simulink model "MotorDriveUnit_Component_harness_model"  (R2023a)
settings: Solver=daessc  StartTime=0.0  StopTime=600  RelTol=1e-3
PreLoadFcn:
  | MotorDriveUnit_Component_harness_params
undefined symbols (not defined in the file or in its folder): batteryHighVoltage, initial, Minus, motorDriveUnit, Plus
libraries: fl_lib x24, nesl_utility x11, sdl_lib x1
settings Model: Creator=isaacito  LastModifiedBy=isaacito
settings DataIOCC: DSMLogging=off
settings OptimizationCC: ReuseModelBlockBuffer=off
settings ModelReferenceCC: EnableRefExpFcnMdlSchedulingChecks=on
settings SimscapeCC: SimscapeLogType=all  SimscapeLogSimulationStatistics=on  SimscapeLogLimitData=off

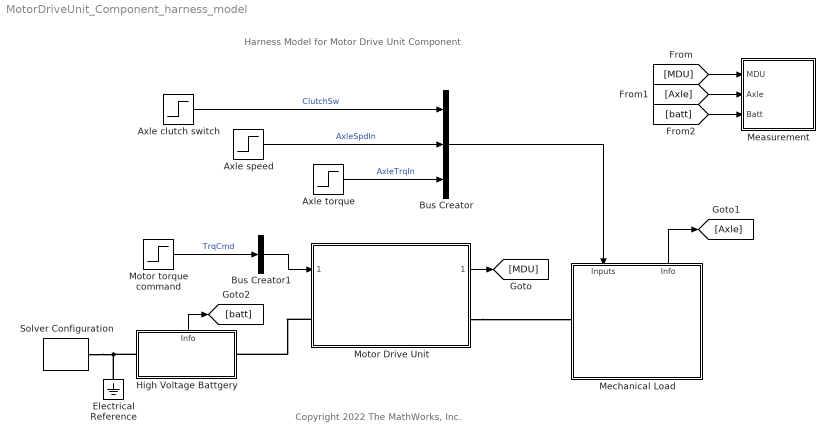
== system MotorDriveUnit_Component_harness_model ==
  note: Harness Model for Motor Drive Unit Component
  note: Copyright 2022 The MathWorks, Inc.
  Axle clutch switch : Step  After=0  SampleTime=0
      settings: AttributesFormatString=|
      | Before %<Before>
      | Time %<Time>
      | After %<After>
  Axle speed : Step  After=0  SampleTime=0
      settings: AttributesFormatString=|
      | Before %<Before>
      | Time %<Time>
      | After %<After>
  Axle torque : Step  Time=400  Before=-10  After=0  SampleTime=0
      settings: AttributesFormatString=|
      | Before %<Before>
      | Time %<Time>
      | After %<After>
  Bus Creator : BusCreator  Inputs=3
  Bus Creator1 : BusCreator  Inputs=1
  Electrical Reference : fl_lib/Electrical/Electrical Elements/Electrical Reference
  High Voltage Battgery : Subsystem
      settings: PortSchema="{\"entries\":[{\"content\":{\"sides\":[{\"content\":{\"connectorIds\":[\"LConn1\"]},\"type\":\"ConnectorPlacement.EquallySpacedRectSide\",\"uuid\":\"8acd7e9a-bb08-4de6-aa14-0989ebba81b9\"},{\"content\":{\"connectorIds\":[\"RConn1\"],\"side\":\"RIGHT\"},\"type\":\"ConnectorPlacement.EquallySpacedRectSide\",\"uuid\":\"f80e1afc-966f-4d6b-84f9-f0b60dd6f20c\"},{\"content\":{\"connectorIds\":[\"Out1\"],\"side\":\"TOP\"},\"type\":\"ConnectorPlacement.EquallySpacedRectSide\",\"uuid\":\"52ccb2b1-bd5e-4dcb-b9b6-0ef03b912c33\"}]},\"type\":\"ConnectorPlacement.EquallySpacedConnector\",\"uuid\":\"b55f48a4-f283-4a77-8513-99b31abb285a\"}],\"packageUris\":[\"http://schema.mathworks.com/mf0/Connector/R2020b\"],\"version\":\"1.0\"}"
  Measurement : Subsystem
  Mechanical Load : Subsystem
      settings: PortSchema="{\"entries\":[{\"content\":{\"sides\":[{\"content\":{\"connectorIds\":[\"LConn1\"]},\"type\":\"ConnectorPlacement.EquallySpacedRectSide\",\"uuid\":\"18221845-08ef-4cf2-b090-320221152030\"},{\"content\":{\"connectorIds\":[],\"side\":\"RIGHT\"},\"type\":\"ConnectorPlacement.EquallySpacedRectSide\",\"uuid\":\"d5b0548b-74c8-455a-9783-7dc299f3571f\"},{\"content\":{\"connectorIds\":[\"In1\",\"Out1\"],\"side\":\"TOP\"},\"type\":\"ConnectorPlacement.EquallySpacedRectSide\",\"uuid\":\"542d8e55-6d7f-4c9a-9fdc-66897ed9f466\"}]},\"type\":\"ConnectorPlacement.EquallySpacedConnector\",\"uuid\":\"3cd4c536-0337-4305-a842-969bfb1fefe3\"}],\"packageUris\":[\"http://schema.mathworks.com/mf0/Connector/R2020b\"],\"version\":\"1.0\"}"
  Motor Drive Unit : Subsystem  ReferencedSubsystem=MotorDriveUnit_refsub_Basic  torque_max=motorDriveUnit.trqMax_Nm  Value=motorDriveUnit.powerMax_kW  Tc=motorDriveUnit.responseTime_s  eff=motorDriveUnit.efficiency_pct  w_eff=motorDriveUnit.spd_eff_rpm  T_eff=motorDriveUnit.trq_eff_Nm  thermal_mass=motorDriveUnit.thermalMass_J_perK  temperature=initial.MDU_Temperature_K  k=motorDriveUnit.dampSpringStiffness_Nm_per_rad  mu_visc=motorDriveUnit.dampSpringFriction_Nm_per_rpm  w_tol=smoothing.MDU_dampSpringVelTol_rpm  T=initial.MDU_AirTemp_K
      settings: PortSchema="{\"entries\":[{\"content\":{\"sides\":[{\"content\":{\"connectorIds\":[\"In1\",\"LConn1\"]},\"type\":\"ConnectorPlacement.EquallySpacedRectSide\",\"uuid\":\"02d16a10-ccfb-4288-a5a1-1144159c5ca2\"},{\"content\":{\"connectorIds\":[\"Out1\",\"LConn2\"],\"side\":\"RIGHT\"},\"type\":\"ConnectorPlacement.EquallySpacedRectSide\",\"uuid\":\"b2601986-efe5-4f5e-bd54-3f5cb03e9252\"},{\"content\":{\"side\":\"TOP\"},\"type\":\"ConnectorPlacement.EquallySpacedRectSide\",\"uuid\":\"248805f0-4416-4f49-8b0b-c2d3fe77e89e\"}]},\"type\":\"ConnectorPlacement.EquallySpacedConnector\",\"uuid\":\"35449164-35fe-478e-9b2e-66e853caa6da\"}],\"packageUris\":[\"http://schema.mathworks.com/mf0/Connector/R2020b\"],\"version\":\"1.0\"}"
  Motor torque command : Step  Time=300  Before=150  After=-50  SampleTime=0
      settings: AttributesFormatString=|
      | Before %<Before>
      | Time %<Time>
      | After %<After>
  Solver Configuration : nesl_utility/Solver Configuration  PhysicalDomain=network_engine_domain  SubClassName=solver  LeftPortType=input  RightPortType=generic  Tones=[]  Harmonics=[]  SimulateNoise=off  Profile=off  UseLocalSampling=off  EnableSwitchedLinearOptims=on  FrequencyDomain=off  UseCCode=off  RelTol=0.001  AbsTol=1e-06  MinStep=1e-09  ToWorkspace=off  RevertToSquareIcSolve=off  NumHomotopyIterations=100  PhasorMode=off  PhasorModeNumHarmonics=1  ConsistencySolver=NEWTON_FTOL  IndexReductionMethod=DerivativeReplacement  DoDC=off  ResidualTolerance=1e-09  ConsistencyTolSource=GLOBAL  ConsistencyAbsTol=0.001  ConsistencyRelTol=0.001  ConsistencyTolFactor=0.001  UseLocalSolver=off  LocalSolverChoice=NE_BACKWARD_EULER_ADVANCER  ResolveIndetEquations=on  FunctionEvalNumThread=1  LocalSolverSampleTime=0.001  DoFixedCost=off  MaxNonlinIter=3  MaxModeIter=2  ComputeImpulses=off  ImpulseIterations=2  LinearAlgebra=auto  LinearAlgebraNumThread=0  EquationFormulation=NE_TIME_EF  DelaysMemoryBudget=1024  AutomaticFiltering=on  FilteringTimeConstant=0.001  PartitionStorageMethod=AS_NEEDED  PartitionMemoryBudget=1024  PartitionMethod=ROBUST
      settings: AttributesFormatString=Local solver %<UseLocalSolver>
  wires:
  Axle speed/1 -> Bus Creator/2  "AxleSpdIn"
  Axle torque/1 -> Bus Creator/3  "AxleTrqIn"
  Motor Drive Unit/1 -> [MDU]
  [MDU] -> Measurement/1(MDU)
  Motor torque command/1 -> Bus Creator1/1  "TrqCmd"
  Bus Creator1/1 -> Motor Drive Unit/1
  [Axle] -> Measurement/2(Axle)
  High Voltage Battgery/1(Info) -> [batt]
  [batt] -> Measurement/3(Batt)
  Bus Creator/1 -> Mechanical Load/1(Inputs)
  Mechanical Load/1(Info) -> [Axle]
  Axle clutch switch/1 -> Bus Creator/1  "ClutchSw"
  connections:
  Motor Drive Unit/LConn1 -- High Voltage Battgery/RConn1
  Electrical Reference/LConn1 -- High Voltage Battgery/LConn1 -- Solver Configuration/RConn1
  Motor Drive Unit/LConn2 -- Mechanical Load/LConn1

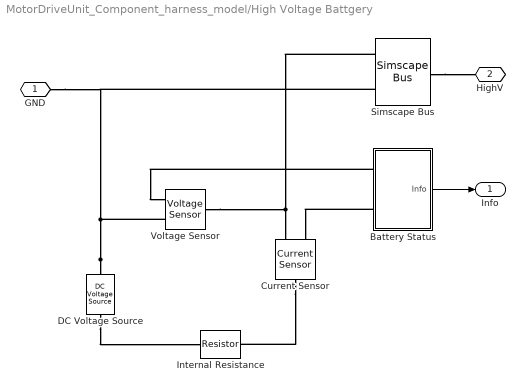
== system MotorDriveUnit_Component_harness_model/High Voltage Battgery ==
  Battery Status : Subsystem
  Current Sensor : fl_lib/Electrical/Electrical Sensors/Current Sensor
  DC Voltage Source : fl_lib/Electrical/Electrical Sources/DC Voltage Source  v0=batteryHighVoltage.voltage_V V
      settings: AttributesFormatString=%<v0> [%<v0_unit>]
  Internal Resistance : fl_lib/Electrical/Electrical Elements/Resistor  R=batteryHighVoltage.internal_R_Ohm Ohm  i_specify=off  i_priority=High  i=0 A  i_nominal_specify=off  i_nominal_unit=A  i_nominal_value=1  v_specify=off  v_priority=High  v=0 V  v_nominal_specify=off  v_nominal_unit=V  v_nominal_value=1
      settings: AttributesFormatString=%<R> [%<R_unit>]
  Simscape Bus : SimscapeBus  HierarchyStrings=Plus;Minus  ConnectionType=Bus: Bus_HighVoltage
      settings: AttributesFormatString=%<ConnectionType>
  Voltage Sensor : fl_lib/Electrical/Electrical Sensors/Voltage Sensor
  GND : PMIOPort  Side=Left
  HighV : PMIOPort  Port=2  Side=Right
  Info : Outport
  wires:
  Battery Status/1(Info) -> Info/1
  connections:
  DC Voltage Source/RConn1 -- Simscape Bus/LConn2 -- GND/RConn1 -- Voltage Sensor/RConn2
  Simscape Bus/LConn1 -- Voltage Sensor/LConn1 -- Current Sensor/RConn2
  Battery Status/LConn2 -- Current Sensor/RConn1
  Simscape Bus/RConn1 -- HighV/RConn1
  Current Sensor/LConn1 -- Internal Resistance/RConn1
  DC Voltage Source/LConn1 -- Internal Resistance/LConn1
  Battery Status/LConn1 -- Voltage Sensor/RConn1

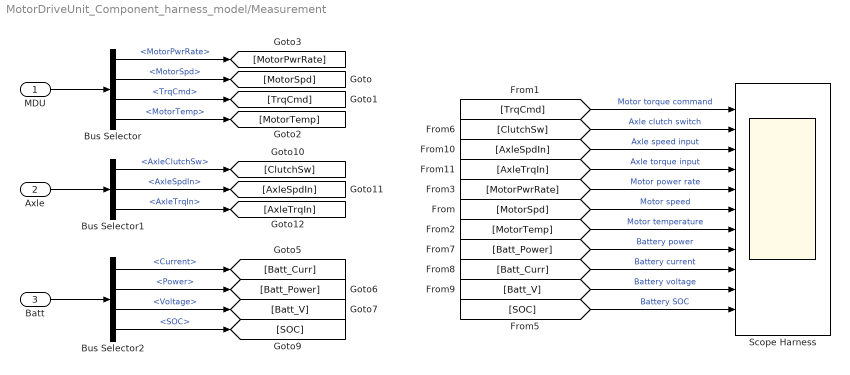
== system MotorDriveUnit_Component_harness_model/Measurement ==
  MDU : Inport
  Axle : Inport  Port=2
  Batt : Inport  Port=3
  Bus Selector : BusSelector  OutputSignals=MotorPwrRate,MotorSpd,TrqCmd,MotorTemp
  Bus Selector1 : BusSelector  OutputSignals=AxleClutchSw,AxleSpdIn,AxleTrqIn
  Bus Selector2 : BusSelector  OutputSignals=Current,Power,Voltage,SOC
  Scope Harness : Scope  NumInputPorts=11
  wires:
  MDU/1 -> Bus Selector/1
  Bus Selector/2 -> [MotorSpd]  "<MotorSpd>"
  Bus Selector/3 -> [TrqCmd]  "<TrqCmd>"
  Bus Selector/4 -> [MotorTemp]  "<MotorTemp>"
  Axle/1 -> Bus Selector1/1
  Bus Selector2/3 -> [Batt_V]  "<Voltage>"
  Bus Selector2/4 -> [SOC]  "<SOC>"
  Bus Selector2/2 -> [Batt_Power]  "<Power>"
  Bus Selector2/1 -> [Batt_Curr]  "<Current>"
  Batt/1 -> Bus Selector2/1
  Bus Selector1/1 -> [ClutchSw]  "<AxleClutchSw>"
  Bus Selector1/2 -> [AxleSpdIn]  "<AxleSpdIn>"
  [TrqCmd] -> Scope Harness/1  "Motor torque command"
  Bus Selector1/3 -> [AxleTrqIn]  "<AxleTrqIn>"
  [ClutchSw] -> Scope Harness/2  "Axle clutch switch"
  [AxleSpdIn] -> Scope Harness/3  "Axle speed input"
  [AxleTrqIn] -> Scope Harness/4  "Axle torque input"
  Bus Selector/1 -> [MotorPwrRate]  "<MotorPwrRate>"
  [MotorPwrRate] -> Scope Harness/5  "Motor power rate"
  [MotorSpd] -> Scope Harness/6  "Motor speed"
  [MotorTemp] -> Scope Harness/7  "Motor temperature"
  [Batt_Power] -> Scope Harness/8  "Battery power"
  [Batt_Curr] -> Scope Harness/9  "Battery current"
  [Batt_V] -> Scope Harness/10  "Battery voltage"
  [SOC] -> Scope Harness/11  "Battery SOC"

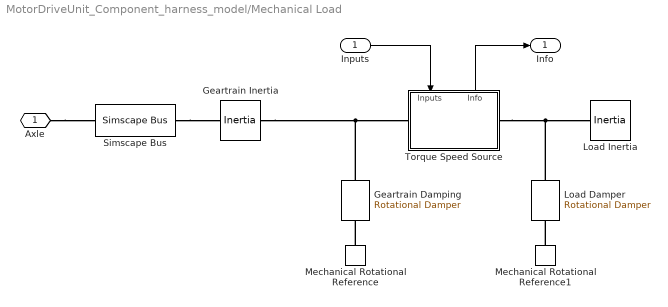
== system MotorDriveUnit_Component_harness_model/Mechanical Load ==
  Inputs : Inport
  Geartrain Damping : fl_lib/Mechanical/Rotational Elements/Rotational Damper  D=0.001 m*N/rpm  w_specify=off  w_priority=None  w=0 rad/s  w_nominal_specify=off  w_nominal_unit=rad/s  w_nominal_value=1  t_specify=off  t_priority=None  t=0 N*m  t_nominal_specify=off  t_nominal_unit=N*m  t_nominal_value=1
      settings: AttributesFormatString=|
      | %<D>
      | %<D_unit>
  Geartrain Inertia : fl_lib/Mechanical/Rotational Elements/Inertia  inertia=15*0.3^2 kg*m^2  num_ports=foundation.enum.numPorts2.two  w_specify=on  w_priority=None  w=0 rpm  w_nominal_specify=off  w_nominal_unit=rad/s  w_nominal_value=1  t_specify=off  t_priority=None  t=0 N*m  t_nominal_specify=off  t_nominal_unit=N*m  t_nominal_value=1
      settings: InternalSimscapePortConfiguration="{\"Bottom\":[],\"Left\":[{\"id\":\"I\",\"label\":\"\",\"type\":\"foundation.mechanical.rotational.rotational\"}],\"Right\":[{\"id\":\"J\",\"label\":\"\",\"type\":\"foundation.mechanical.rotational.rotational\"}],\"Top\":[]}"
      settings: AttributesFormatString=|
      | %<inertia> %<inertia_unit>
      | Priority: %<w_priority>
  Load Damper : fl_lib/Mechanical/Rotational Elements/Rotational Damper  D=0.1 N*m/rpm  w_specify=off  w_priority=None  w=0 rad/s  w_nominal_specify=off  w_nominal_unit=rad/s  w_nominal_value=1  t_specify=off  t_priority=None  t=0 N*m  t_nominal_specify=off  t_nominal_unit=N*m  t_nominal_value=1
      settings: AttributesFormatString=|
      | %<D>
      | %<D_unit>
  Load Inertia : fl_lib/Mechanical/Rotational Elements/Inertia  inertia=2000*0.3^3 kg*m^2  num_ports=foundation.enum.numPorts2.one  w_specify=on  w_priority=High  w=initial.loadInertiaSpd_rpm rpm  w_nominal_specify=off  w_nominal_unit=rad/s  w_nominal_value=1  t_specify=off  t_priority=None  t=0 N*m  t_nominal_specify=off  t_nominal_unit=N*m  t_nominal_value=1
      settings: AttributesFormatString=|
      | %<inertia> [%<inertia_unit>]
      | %<w> [%<w_unit>]
      | Priority: %<w_priority>
  Mechanical Rotational Reference : fl_lib/Mechanical/Rotational Elements/Mechanical Rotational Reference
  Mechanical Rotational Reference1 : fl_lib/Mechanical/Rotational Elements/Mechanical Rotational Reference
  Simscape Bus : SimscapeBus  HierarchyStrings=AngSpd  ConnectionType=Bus: Bus_Rotational
  Torque Speed Source : Subsystem
      settings: PortSchema="{\"entries\":[{\"content\":{\"sides\":[{\"content\":{\"connectorIds\":[\"LConn1\"]},\"type\":\"ConnectorPlacement.EquallySpacedRectSide\",\"uuid\":\"92a06674-aaa2-495f-b380-fd1e5a218eb3\"},{\"content\":{\"connectorIds\":[\"RConn1\"],\"side\":\"RIGHT\"},\"type\":\"ConnectorPlacement.EquallySpacedRectSide\",\"uuid\":\"3e9807eb-b215-4ab1-ac02-6574a58f93c0\"},{\"content\":{\"connectorIds\":[\"In1\",\"Out1\"],\"side\":\"TOP\"},\"type\":\"ConnectorPlacement.EquallySpacedRectSide\",\"uuid\":\"937668c8-63b6-43a7-85c7-81bf7d359316\"}]},\"type\":\"ConnectorPlacement.EquallySpacedConnector\",\"uuid\":\"ba9b6e46-9639-4838-8d50-8636a64d3a24\"}],\"packageUris\":[\"http://schema.mathworks.com/mf0/Connector/R2020b\"],\"version\":\"1.0\"}"
  Axle : PMIOPort  Side=Left
  Info : Outport
  wires:
  Torque Speed Source/1(Info) -> Info/1
  Inputs/1 -> Torque Speed Source/1(Inputs)
  connections:
  Mechanical Rotational Reference/LConn1 -- Geartrain Damping/RConn1
  Mechanical Rotational Reference1/LConn1 -- Load Damper/RConn1
  Simscape Bus/LConn1 -- Geartrain Inertia/RConn1
  Axle/RConn1 -- Simscape Bus/RConn1
  Torque Speed Source/RConn1 -- Load Damper/LConn1 -- Load Inertia/LConn1
  Geartrain Inertia/LConn1 -- Geartrain Damping/LConn1 -- Torque Speed Source/LConn1

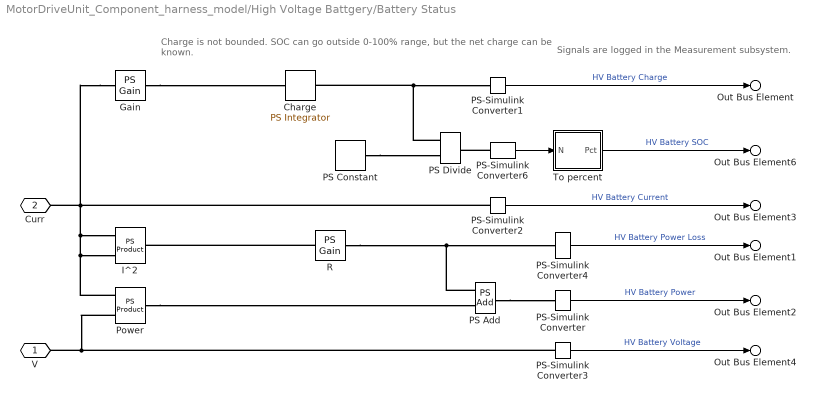
== system MotorDriveUnit_Component_harness_model/High Voltage Battgery/Battery Status ==
  note: Signals are logged in the Measurement subsystem.
  note: Charge is not bounded. SOC can go outside 0-100% range,
      | but the net charge can be known.
  Charge : fl_lib/Physical Signals/Linear Operators/PS Integrator  reset_method=foundation.enum.IntegratorResetSpec.None  initial_condition_spec=foundation.enum.IntegratorICSpec.Internal  saturation_spec=foundation.enum.IntegratorSaturationSpec.None  saturation_source_spec=foundation.enum.IntegratorSaturationSourceSpec.Internal  x0=initial.hvBattery_Charge_Ahr A*hr  xu=inf s  xl=-inf s
      settings: AttributesFormatString=%<x0> [%<x0_unit>]
  Gain : fl_lib/Physical Signals/Functions/PS Gain  gain=-1
      settings: AttributesFormatString=%<gain>
  I^2 : fl_lib/Physical Signals/Functions/PS Product
  PS Add : fl_lib/Physical Signals/Functions/PS Add
  PS Constant : fl_lib/Physical Signals/Sources/PS Constant  constant=batteryHighVoltage.charge_Ahr A*hr
      settings: AttributesFormatString=%<constant> [%<constant_unit>]
  PS Divide : fl_lib/Physical Signals/Functions/PS Divide
  PS-Simulink Converter : nesl_utility/PS-Simulink Converter  PhysicalDomain=network_engine_domain  SubClassName=ps_output  LeftPortType=input  RightPortType=output  PseudoPeriodic=off  Frequencies=[]  VectorFormat=1-D array  Unit=kW  AffineConversion=off
  PS-Simulink Converter1 : nesl_utility/PS-Simulink Converter  PhysicalDomain=network_engine_domain  SubClassName=ps_output  LeftPortType=input  RightPortType=output  PseudoPeriodic=off  Frequencies=[]  VectorFormat=1-D array  Unit=A*hr  AffineConversion=off
  PS-Simulink Converter2 : nesl_utility/PS-Simulink Converter  PhysicalDomain=network_engine_domain  SubClassName=ps_output  LeftPortType=input  RightPortType=output  PseudoPeriodic=off  Frequencies=[]  VectorFormat=1-D array  Unit=A  AffineConversion=off
  PS-Simulink Converter3 : nesl_utility/PS-Simulink Converter  PhysicalDomain=network_engine_domain  SubClassName=ps_output  LeftPortType=input  RightPortType=output  PseudoPeriodic=off  Frequencies=[]  VectorFormat=1-D array  Unit=V  AffineConversion=off
  PS-Simulink Converter4 : nesl_utility/PS-Simulink Converter  PhysicalDomain=network_engine_domain  SubClassName=ps_output  LeftPortType=input  RightPortType=output  PseudoPeriodic=off  Frequencies=[]  VectorFormat=1-D array  Unit=W  AffineConversion=off
  PS-Simulink Converter6 : nesl_utility/PS-Simulink Converter  PhysicalDomain=network_engine_domain  SubClassName=ps_output  LeftPortType=input  RightPortType=output  PseudoPeriodic=off  Frequencies=[]  VectorFormat=1-D array  Unit=1  AffineConversion=off
  Power : fl_lib/Physical Signals/Functions/PS Product
  R : fl_lib/Physical Signals/Functions/PS Gain  gain=batteryHighVoltage.internal_R_Ohm Ohm
      settings: AttributesFormatString=%<gain> [%<gain_unit>]
  To percent : Subsystem
  V : PMIOPort  Side=Left
  Curr : PMIOPort  Port=2  Side=Left
  Out Bus Element : Outport  PortName=Info  Element=Charge
      settings: AttributesFormatString=%<Unit>
  Out Bus Element3 : Outport  PortName=Info  Element=Current
      settings: AttributesFormatString=%<Unit>
  Out Bus Element1 : Outport  PortName=Info  Element=PowerLoss
      settings: AttributesFormatString=%<Unit>
  Out Bus Element2 : Outport  PortName=Info  Element=Power
      settings: AttributesFormatString=%<Unit>
  Out Bus Element4 : Outport  PortName=Info  Element=Voltage
      settings: AttributesFormatString=%<Unit>
  Out Bus Element6 : Outport  PortName=Info  Element=SOC
      settings: AttributesFormatString=%<Unit>
  wires:
  PS-Simulink Converter6/1 -> To percent/1(N)
  To percent/1(Pct) -> Out Bus Element6/1  "HV Battery SOC"
  PS-Simulink Converter3/1 -> Out Bus Element4/1  "HV Battery Voltage"
  PS-Simulink Converter2/1 -> Out Bus Element3/1  "HV Battery Current"
  PS-Simulink Converter4/1 -> Out Bus Element1/1  "HV Battery Power Loss"
  PS-Simulink Converter1/1 -> Out Bus Element/1  "HV Battery Charge"
  PS-Simulink Converter/1 -> Out Bus Element2/1  "HV Battery Power"
  connections:
  PS-Simulink Converter6/LConn1 -- PS Divide/RConn1
  Power/RConn1 -- PS Add/LConn2
  PS Constant/RConn1 -- PS Divide/LConn2
  PS Add/RConn1 -- PS-Simulink Converter/LConn1
  R/LConn1 -- I^2/RConn1
  PS Divide/LConn1 -- PS-Simulink Converter1/LConn1 -- Charge/RConn1
  Gain/RConn1 -- Charge/LConn1
  PS Add/LConn1 -- PS-Simulink Converter4/LConn1 -- R/RConn1
  Power/LConn1 -- PS-Simulink Converter3/LConn1 -- V/RConn1
  Gain/LConn1 -- PS-Simulink Converter2/LConn1 -- Curr/RConn1 -- I^2/LConn1 -- Power/LConn2 -- I^2/LConn2

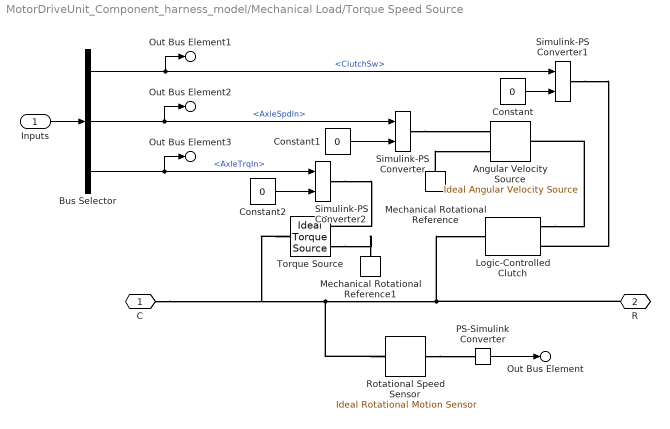
== system MotorDriveUnit_Component_harness_model/Mechanical Load/Torque Speed Source ==
  Inputs : Inport
  Angular Velocity Source : fl_lib/Mechanical/Mechanical Sources/Ideal Angular Velocity Source
  Bus Selector : BusSelector  OutputSignals=ClutchSw,AxleSpdIn,AxleTrqIn
  Constant : Constant  Value=0
  Constant1 : Constant  Value=0
  Constant2 : Constant  Value=0
  Logic-Controlled Clutch : sdl_lib/Clutches/Logic-Controlled Clutch  transition_model=sdl.enum.transitionModel.instant  transition_time_constant=0.1 s  t_friction=5000 N*m  t_locked=5000 N*m  w_tol=0.1 rpm  initial_state_locked=sdl.enum.initial_lock.unlocked
      settings: InternalSimscapePortConfiguration="{\"Bottom\":[],\"Left\":[{\"id\":\"E\",\"label\":\"E\",\"type\":\"input\"},{\"id\":\"B\",\"label\":\"B\",\"type\":\"foundation.mechanical.rotational.rotational\"}],\"Right\":[{\"id\":\"F\",\"label\":\"F\",\"type\":\"foundation.mechanical.rotational.rotational\"}],\"Top\":[]}"
  Mechanical Rotational Reference : fl_lib/Mechanical/Rotational Elements/Mechanical Rotational Reference
  Mechanical Rotational Reference1 : fl_lib/Mechanical/Rotational Elements/Mechanical Rotational Reference
  PS-Simulink Converter : nesl_utility/PS-Simulink Converter  PhysicalDomain=network_engine_domain  SubClassName=ps_output  LeftPortType=input  RightPortType=output  PseudoPeriodic=off  Frequencies=[]  VectorFormat=inherit  Unit=rpm  AffineConversion=off
  Rotational Speed Sensor : fl_lib/Mechanical/Mechanical Sensors/Ideal Rotational Motion Sensor  reference=foundation.enum.MeasurementReference.absolute  acceleration_port=false  velocity_port=true  position_port=false  wrap_angle=simscape.enum.onoff.off  offset=0 rad
      settings: InternalSimscapePortConfiguration="{\"Bottom\":[],\"Left\":[{\"id\":\"R\",\"label\":\"R\",\"type\":\"foundation.mechanical.rotational.rotational\"}],\"Right\":[{\"id\":\"W\",\"label\":\"W\",\"type\":\"output\"}],\"Top\":[]}"
  Simulink-PS Converter : nesl_utility/Simulink-PS Converter  PhysicalDomain=network_engine_domain  SubClassName=ps_input  LeftPortType=input  RightPortType=output  PseudoPeriodic=off  Frequencies=[]  NoiseDistribution=none  NoiseParameters=[]  Unit=rpm  AffineConversion=off  FilteringAndDerivatives=provide  SimscapeFilterOrder=1  InputFilterTimeConstant=0.001  UdotUserProvided=1
  Simulink-PS Converter1 : nesl_utility/Simulink-PS Converter  PhysicalDomain=network_engine_domain  SubClassName=ps_input  LeftPortType=input  RightPortType=output  PseudoPeriodic=off  Frequencies=[]  NoiseDistribution=none  NoiseParameters=[]  Unit=1  AffineConversion=off  FilteringAndDerivatives=provide  SimscapeFilterOrder=1  InputFilterTimeConstant=0.001  UdotUserProvided=1
      settings: AttributesFormatString=|
      | %<Unit>
      | Derivative: %<FilteringAndDerivatives>
  Simulink-PS Converter2 : nesl_utility/Simulink-PS Converter  PhysicalDomain=network_engine_domain  SubClassName=ps_input  LeftPortType=input  RightPortType=output  PseudoPeriodic=off  Frequencies=[]  NoiseDistribution=none  NoiseParameters=[]  Unit=N*m  AffineConversion=off  FilteringAndDerivatives=provide  SimscapeFilterOrder=1  InputFilterTimeConstant=0.001  UdotUserProvided=1
  Torque Source : fl_lib/Mechanical/Mechanical Sources/Ideal Torque Source
  C : PMIOPort  Side=Left
  R : PMIOPort  Port=2  Side=Right
  Out Bus Element : Outport  PortName=Info  Element=AxleSpd
  Out Bus Element1 : Outport  PortName=Info  Element=AxleClutchSw
  Out Bus Element2 : Outport  PortName=Info  Element=AxleSpdIn
  Out Bus Element3 : Outport  PortName=Info  Element=AxleTrqIn
  wires:
  Inputs/1 -> Bus Selector/1
  Bus Selector/1 -> Simulink-PS Converter1/1, Out Bus Element1/1  "<ClutchSw>"
  Bus Selector/2 -> Simulink-PS Converter/1, Out Bus Element2/1  "<AxleSpdIn>"
  Bus Selector/3 -> Simulink-PS Converter2/1, Out Bus Element3/1  "<AxleTrqIn>"
  PS-Simulink Converter/1 -> Out Bus Element/1
  Constant/1 -> Simulink-PS Converter1/2
  Constant1/1 -> Simulink-PS Converter/2
  Constant2/1 -> Simulink-PS Converter2/2
  connections:
  Simulink-PS Converter/RConn1 -- Angular Velocity Source/RConn1
  Mechanical Rotational Reference/LConn1 -- Angular Velocity Source/RConn2
  Logic-Controlled Clutch/LConn2 -- Angular Velocity Source/LConn1
  Simulink-PS Converter1/RConn1 -- Logic-Controlled Clutch/LConn1
  Rotational Speed Sensor/LConn1 -- R/RConn1 -- Logic-Controlled Clutch/RConn1 -- C/RConn1 -- Torque Source/LConn1
  Rotational Speed Sensor/RConn1 -- PS-Simulink Converter/LConn1
  Simulink-PS Converter2/RConn1 -- Torque Source/RConn1
  Torque Source/RConn2 -- Mechanical Rotational Reference1/LConn1

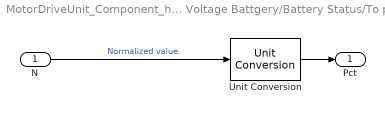
== system MotorDriveUnit_Component_harness_model/High Voltage Battgery/Battery Status/To percent ==
  N : Inport
  Unit Conversion : UnitConversion
  Pct : Outport  Unit=%
      settings: AttributesFormatString=%<Unit>
  wires:
  N/1 -> Unit Conversion/1  "Normalized value"
  Unit Conversion/1 -> Pct/1
